simulink model "afe_inv_psm_param"  (R2026b)
settings: Solver=ode23t  StopTime=param.sim.simlength  FixedStep=tc  MaxStep=param.glb_time.tc  RelTol=1e-4
values from neighbouring files (symbols this model uses):
  param = add_template_extras(param, options)    [init_model.m]
undefined symbols (not defined in the file or in its folder): magnitude, omega_m_bez
libraries: fl_lib x330, nesl_utility x174, igbt_simple_2th_lib x12, moving_average_filter x10, moving_average_filter_cc x8, sl_discontinuities x3, single_phase_transformer_lib x3, linear_double_integrator_observer_ccaller x2, discrete_time_low_pass_filter x2, threephase_inductor_lib x2, three_phase_pwm_modulator x2, three_phase_inverter_ideal_switch_based_model x2
(part 7 of 13)

== system afe_inv_psm_param/afe_abc_inv_psm_mod1/AFE_control/afe_control/grid_current_sequences_and_reactive_pwr_ctrl/sequences_current_control/Positive-Seq. eta-Control ==
  ff : Inport
  e : Inport  Port=2
  1/Ti : Gain  Gain=param.afe.ctrl.kp_rc_pos_grid  SaturateOnIntegerOverflow=on  OutDataTypeStr=Inherit: Same as input  ParamDataTypeStr=Inherit: Same as input
  Saturation : Saturate  UpperLimit=param.afe.ctrl.ieta_pos_ref_lim  LowerLimit=-param.afe.ctrl.ieta_pos_ref_lim
  Sum : Sum  Inputs=|++
  Sum2 : Sum  Inputs=+++  SaturateOnIntegerOverflow=on
  Sum3 : Sum  Inputs=-+  SaturateOnIntegerOverflow=on
  Unit Delay4 : UnitDelay  SampleTime=-1
  kp : Gain  Gain=param.afe.ctrl.ki_rc_pos_grid*param.glb_time.ts_afe  SaturateOnIntegerOverflow=on  OutDataTypeStr=Inherit: Same as input  ParamDataTypeStr=Inherit: Same as input
  u : Outport  VectorParamsAs1DForOutWhenUnconnected=off
  wires:
  Unit Delay4/1 -> Sum2/3
  Sum3/1 -> Unit Delay4/1
  kp/1 -> Sum2/2
  Sum2/1 -> Saturation/1
  1/Ti/1 -> Sum2/1, Sum3/1
  Saturation/1 -> Sum/1, Sum3/2
  Sum/1 -> u/1
  e/1 -> 1/Ti/1, kp/1  "e"
  ff/1 -> Sum/2

== system afe_inv_psm_param/afe_abc_inv_psm_mod1/AFE_control/afe_control/grid_voltage_phase_lock_loops/FHT-PLL/pll_stageA ==
  gamma_grid : Inport
  ug_abc_pu : Inport  Port=2
  Demux : Demux  Outputs=3
  Math Function : Math  Operator=magnitude^2  SignedPower=on
  Math Function1 : Math  Operator=magnitude^2  SignedPower=on
  Reciprocal Sqrt : Sqrt  Operator=rSqrt
  Saturation : Saturate  UpperLimit=inf  LowerLimit=0.02
  Sum : Sum  Inputs=|++
  filter_and_transformation : Subsystem
  sequences : Subsystem
  u_grid_xi : Outport  VectorParamsAs1DForOutWhenUnconnected=off
  u_grid_eta : Outport  Port=2  VectorParamsAs1DForOutWhenUnconnected=off
  tag scope: Vgrid_unorm_fht=scoped
  wires:
  gamma_grid/1 -> sequences/3(phase_angle)
  sequences/2(u_grid_eta) -> u_grid_eta/1
  sequences/1(u_grid_xi) -> u_grid_xi/1
  ug_abc_pu/1 -> Demux/1
  Demux/1 -> filter_and_transformation/1(ug_a)
  Demux/2 -> filter_and_transformation/2(ug_b)
  Demux/3 -> filter_and_transformation/3(ug_c)
  filter_and_transformation/1(ug_alpha) -> Math Function/1, sequences/1(u_grid_alpha)
  filter_and_transformation/2(ug_beta) -> Math Function1/1, sequences/2(u_grid_beta)
  Math Function/1 -> Sum/1
  Math Function1/1 -> Sum/2
  Sum/1 -> Saturation/1
  Reciprocal Sqrt/1 -> [Vgrid_unorm_fht]
  Saturation/1 -> Reciprocal Sqrt/1

== system afe_inv_psm_param/afe_abc_inv_psm_mod1/AFE_control/afe_control/grid_voltage_phase_lock_loops/FHT-PLL/pll_stageB ==
  u_grid_pos_xi : Inport
  u_grid_pos_eta : Inport  Port=2
  Constant4 : Constant  Value=param.grid.emu.omega_grid_nom
  Gain : Gain  Gain=-1
  Product : Product  RndMeth=Zero
  Product1 : Product  RndMeth=Zero
  Product2 : Product  RndMeth=Zero
  Sum3 : Sum  SaturateOnIntegerOverflow=on
  Sum4 : Sum  SaturateOnIntegerOverflow=on
  Sum5 : Sum  Inputs=++|
  Terminator : Terminator
  Unit Delay1 : UnitDelay  SampleTime=-1
  Unit Delay2 : UnitDelay  SampleTime=-1
  Unit Delay4 : UnitDelay  SampleTime=-1
  bounder1 : MATLAB Function  TreatAsAtomicUnit=on
  double_integrator_observer : Subsystem
  kp : Gain  Gain=param.afe.ctrl.pll_i1_fht*param.glb_time.ts_afe  SaturateOnIntegerOverflow=on  OutDataTypeStr=Inherit: Same as input  ParamDataTypeStr=Inherit: Same as input
  kp1 : Gain  Gain=param.afe.ctrl.pll_p_fht  SaturateOnIntegerOverflow=on  OutDataTypeStr=Inherit: Same as input  ParamDataTypeStr=Inherit: Same as input
  kp2 : Gain  Gain=param.glb_time.ts_afe  SaturateOnIntegerOverflow=on  OutDataTypeStr=Inherit: Same as input  ParamDataTypeStr=Inherit: Same as input
  kp3 : Gain  Gain=1/param.grid.emu.omega_grid_nom  SaturateOnIntegerOverflow=on  OutDataTypeStr=Inherit: Same as input  ParamDataTypeStr=Inherit: Same as input
  gamma_grid_ddsrf_pll : Outport  VectorParamsAs1DForOutWhenUnconnected=off
  omega_grid_ddsrf_pll : Outport  Port=2  VectorParamsAs1DForOutWhenUnconnected=off
  wires:
  Gain/1 -> kp/1, kp1/1
  Product1/1 -> Gain/1
  kp3/1 -> omega_grid_ddsrf_pll/1
  Product/1 -> Terminator/1
  double_integrator_observer/1(omega_hat) -> kp3/1
  Unit Delay4/1 -> Sum3/2
  Sum4/1 -> bounder1/1(u)
  Unit Delay1/1 -> Sum4/2
  Sum3/1 -> Sum5/2, Unit Delay4/1  "i1"
  kp2/1 -> Sum4/1
  Constant4/1 -> Product2/2
  [Vgrid_unorm_fht] -> Product/2, Product1/2
  kp/1 -> Sum3/1
  Sum5/1 -> Product2/1
  bounder1/1(y) -> Unit Delay2/1, Unit Delay1/1
  u_grid_pos_xi/1 -> Product/1
  u_grid_pos_eta/1 -> Product1/1
  Product2/1 -> kp2/1
  kp1/1 -> Sum5/1
  Unit Delay2/1 -> double_integrator_observer/1(theta), gamma_grid_ddsrf_pll/1

== system afe_inv_psm_param/afe_abc_inv_psm_mod1/AFE_control/afe_control/grid_voltage_phase_lock_loops/FHT-PLL_simulink/pll_stageA ==
  gamma_grid : Inport
  ug_abc_pu : Inport  Port=2
  Demux : Demux  Outputs=3
  Math Function : Math  Operator=magnitude^2  SignedPower=on
  Math Function1 : Math  Operator=magnitude^2  SignedPower=on
  Reciprocal Sqrt : Sqrt  Operator=rSqrt
  Saturation : Saturate  UpperLimit=inf  LowerLimit=0.02
  Sum : Sum  Inputs=|++
  filter_and_transformation : Subsystem
  sequences : Subsystem
  u_grid_xi : Outport  VectorParamsAs1DForOutWhenUnconnected=off
  u_grid_eta : Outport  Port=2  VectorParamsAs1DForOutWhenUnconnected=off
  tag scope: Vgrid_unorm_fht_simulink=scoped
  wires:
  Saturation/1 -> Reciprocal Sqrt/1
  Reciprocal Sqrt/1 -> [Vgrid_unorm_fht_simulink]
  Sum/1 -> Saturation/1
  Math Function1/1 -> Sum/2
  Math Function/1 -> Sum/1
  filter_and_transformation/2(ug_beta) -> sequences/2(u_grid_beta), Math Function1/1
  filter_and_transformation/1(ug_alpha) -> sequences/1(u_grid_alpha), Math Function/1
  Demux/3 -> filter_and_transformation/3(ug_c)
  Demux/2 -> filter_and_transformation/2(ug_b)
  Demux/1 -> filter_and_transformation/1(ug_a)
  ug_abc_pu/1 -> Demux/1
  sequences/1(u_grid_xi) -> u_grid_xi/1
  sequences/2(u_grid_eta) -> u_grid_eta/1
  gamma_grid/1 -> sequences/3(phase_angle)

== system afe_inv_psm_param/afe_abc_inv_psm_mod1/AFE_control/afe_control/grid_voltage_phase_lock_loops/FHT-PLL_simulink/pll_stageB ==
  u_grid_pos_xi : Inport
  u_grid_pos_eta : Inport  Port=2
  Constant4 : Constant  Value=param.grid.emu.omega_grid_nom
  Gain : Gain  Gain=-1
  Product : Product  RndMeth=Zero
  Product1 : Product  RndMeth=Zero
  Product2 : Product  RndMeth=Zero
  Sum3 : Sum  SaturateOnIntegerOverflow=on
  Sum4 : Sum  SaturateOnIntegerOverflow=on
  Sum5 : Sum  Inputs=++|
  Terminator : Terminator
  Unit Delay1 : UnitDelay  SampleTime=-1
  Unit Delay2 : UnitDelay  SampleTime=-1
  Unit Delay4 : UnitDelay  SampleTime=-1
  bounder1 : MATLAB Function  TreatAsAtomicUnit=on
  double_integrator_observer : Subsystem
  kp : Gain  Gain=param.afe.ctrl.pll_i1_fht*param.glb_time.ts_afe  SaturateOnIntegerOverflow=on  OutDataTypeStr=Inherit: Same as input  ParamDataTypeStr=Inherit: Same as input
  kp1 : Gain  Gain=param.afe.ctrl.pll_p_fht  SaturateOnIntegerOverflow=on  OutDataTypeStr=Inherit: Same as input  ParamDataTypeStr=Inherit: Same as input
  kp2 : Gain  Gain=param.glb_time.ts_afe  SaturateOnIntegerOverflow=on  OutDataTypeStr=Inherit: Same as input  ParamDataTypeStr=Inherit: Same as input
  kp3 : Gain  Gain=1/param.grid.emu.omega_grid_nom  SaturateOnIntegerOverflow=on  OutDataTypeStr=Inherit: Same as input  ParamDataTypeStr=Inherit: Same as input
  gamma_grid_ddsrf_pll : Outport  VectorParamsAs1DForOutWhenUnconnected=off
  omega_grid_ddsrf_pll : Outport  Port=2  VectorParamsAs1DForOutWhenUnconnected=off
  wires:
  Unit Delay2/1 -> gamma_grid_ddsrf_pll/1, double_integrator_observer/1(theta)
  kp1/1 -> Sum5/1
  Product2/1 -> kp2/1
  u_grid_pos_eta/1 -> Product1/1
  u_grid_pos_xi/1 -> Product/1
  bounder1/1(y) -> Unit Delay1/1, Unit Delay2/1
  Sum5/1 -> Product2/1
  kp/1 -> Sum3/1
  [Vgrid_unorm_fht_simulink] -> Product1/2, Product/2
  Constant4/1 -> Product2/2
  kp2/1 -> Sum4/1
  Sum3/1 -> Unit Delay4/1, Sum5/2  "i1"
  Unit Delay1/1 -> Sum4/2
  Sum4/1 -> bounder1/1(u)
  Unit Delay4/1 -> Sum3/2
  double_integrator_observer/1(omega_hat) -> kp3/1
  Product/1 -> Terminator/1
  kp3/1 -> omega_grid_ddsrf_pll/1
  Product1/1 -> Gain/1
  Gain/1 -> kp1/1, kp/1

== system afe_inv_psm_param/afe_abc_inv_psm_mod1/AFE_control/afe_control/grid_voltage_phase_lock_loops/dq_pll/pll_stageA ==
  phase_grid : Inport
  ug_abc : Inport  Port=2
  Demux : Demux  Outputs=3
  Math Function : Math  Operator=magnitude^2  SignedPower=on
  Math Function1 : Math  Operator=magnitude^2  SignedPower=on
  Reciprocal Sqrt : Sqrt  Operator=rSqrt
  Saturation : Saturate  UpperLimit=inf  LowerLimit=0.02
  Sum : Sum  Inputs=|++
  mormalization_and_transformation : Subsystem
  sequences : Subsystem
  u_grid_pos_xi : Outport  VectorParamsAs1DForOutWhenUnconnected=off
  u_grid_pos_eta : Outport  Port=2  VectorParamsAs1DForOutWhenUnconnected=off
  tag scope: Vgrid_unorm_dqpll=scoped
  wires:
  ug_abc/1 -> Demux/1
  Demux/1 -> mormalization_and_transformation/1(ug_a)
  Demux/2 -> mormalization_and_transformation/2(ug_b)
  Demux/3 -> mormalization_and_transformation/3(ug_c)
  phase_grid/1 -> sequences/3(gamma_grid)
  sequences/1(u_grid_pos_xi) -> u_grid_pos_xi/1
  sequences/2(u_grid_pos_eta) -> u_grid_pos_eta/1
  Math Function1/1 -> Sum/2
  mormalization_and_transformation/1(ug_alpha) -> Math Function/1, sequences/1(u_grid_alpha)
  mormalization_and_transformation/2(ug_beta) -> Math Function1/1, sequences/2(u_grid_beta)
  Reciprocal Sqrt/1 -> [Vgrid_unorm_dqpll]
  Sum/1 -> Saturation/1
  Math Function/1 -> Sum/1
  Saturation/1 -> Reciprocal Sqrt/1

== system afe_inv_psm_param/afe_abc_inv_psm_mod1/AFE_control/afe_control/grid_voltage_phase_lock_loops/dq_pll/pll_stageB ==
  u_grid_pos_xi : Inport
  u_grid_pos_eta : Inport  Port=2
  -2<x<2 : Saturate  UpperLimit=2  LowerLimit=-2
  Constant4 : Constant  Value=param.grid.emu.omega_grid_nom
  Gain : Gain  Gain=1/param.grid.emu.omega_grid_nom
  Product1 : Product  RndMeth=Zero
  Product2 : Product  RndMeth=Zero
  Sum3 : Sum  SaturateOnIntegerOverflow=on
  Sum4 : Sum  SaturateOnIntegerOverflow=on
  Sum5 : Sum  Inputs=++|
  Terminator : Terminator
  Unit Delay1 : UnitDelay  SampleTime=-1
  Unit Delay2 : UnitDelay  SampleTime=-1
  Unit Delay4 : UnitDelay  SampleTime=-1
  bounder1 : MATLAB Function  TreatAsAtomicUnit=on
  double_integrator_observer : Subsystem
  kp : Gain  Gain=param.afe.ctrl.pll_i1*param.glb_time.ts_afe  SaturateOnIntegerOverflow=on  OutDataTypeStr=Inherit: Same as input  ParamDataTypeStr=Inherit: Same as input
  kp2 : Gain  Gain=param.glb_time.ts_afe  SaturateOnIntegerOverflow=on  OutDataTypeStr=Inherit: Same as input  ParamDataTypeStr=Inherit: Same as input
  scheduled-p-gain : Subsystem
      settings: PortSchema="{\"entries\":[{\"content\":{\"sides\":[{\"content\":{},\"type\":\"ConnectorPlacement.EquallySpacedRectSide\",\"uuid\":\"88e64df2-a299-4c1b-9bac-7a615cd04a00\"},{\"content\":{\"side\":\"RIGHT\"},\"type\":\"ConnectorPlacement.EquallySpacedRectSide\",\"uuid\":\"ef1d7318-b0e2-4e96-bf99-c42bb4ec5202\"},{\"content\":{\"connectorIds\":[\"In1\"],\"side\":\"TOP\"},\"type\":\"ConnectorPlacement.EquallySpacedRectSide\",\"uuid\":\"96582c59-f6c8-40f1-b3cf-394cc239c4b2\"},{\"content\":{\"connectorIds\":[\"Out1\"],\"side\":\"BOTTOM\"},\"type\":\"ConnectorPlacement.EquallySpacedRectSide\",\"uuid\":\"9ac5cd0d-958f-4b67-b4ea-90856a0aa038\"}]},\"type\":\"ConnectorPlacement.EquallySpacedConnector\",\"uuid\":\"ca37db80-6b94-4315-bd9c-66307567cd1f\"}],\"packageUris\":[\"http://schema.mathworks.com/mf0/Connector/R2020b\"],\"version\":\"1.0\"}"
  phase_grid_pll : Outport  VectorParamsAs1DForOutWhenUnconnected=off
  omega_grid_pu_pll : Outport  Port=2  VectorParamsAs1DForOutWhenUnconnected=off
  wires:
  Unit Delay4/1 -> Sum3/2
  Sum3/1 -> -2<x<2/1
  Sum4/1 -> bounder1/1(u)
  Unit Delay1/1 -> Sum4/2
  -2<x<2/1 -> Sum5/2, Unit Delay4/1  "i1"
  kp2/1 -> Sum4/1
  Constant4/1 -> Product2/2
  [Vgrid_unorm_dqpll] -> Product1/2
  kp/1 -> Sum3/1
  Sum5/1 -> Product2/1
  bounder1/1(y) -> Unit Delay1/1, Unit Delay2/1
  u_grid_pos_eta/1 -> Product1/1
  Product2/1 -> kp2/1
  Product1/1 -> scheduled-p-gain/1(In1), kp/1
  scheduled-p-gain/1(Out2) -> Sum5/1
  Unit Delay2/1 -> double_integrator_observer/1(phase), phase_grid_pll/1
  double_integrator_observer/1(omega_hat) -> Gain/1
  Gain/1 -> omega_grid_pu_pll/1
  u_grid_pos_xi/1 -> Terminator/1

== system afe_inv_psm_param/afe_abc_inv_psm_mod1/AFE_control/afe_control/grid_voltage_phase_lock_loops/dq_pll_ccaller/first_harmonic_tracker_phase_u ==
  u : Inport
  Bus Selector : BusSelector  OutputSignals=output_pu_hat
  C Caller : CCaller  FunctionName=first_harmonic_tracker_process_simulink  PortSpecificationStruct="%)30     .    B \\   8    (     @         %    \"     D    !     0         %  0 \"0    $    _    07)G3F%M90  4&]R=$YA;64 4V-O<&4     26YD97@     5'EP90      4VEZ90      27-';&]B86P   X    P    !@    @    $          4    (     0    ,    !         !   P!O=70 #@   #     &    \"     0         !0    @    !     P    $         $  # &]U=  .    .     8    (    !          %    \"     $    &     0         0  ...(+4988 chars)"
  Constant : Constant  Value=param.glb_time.ts_afe
  Constant1 : Constant  Value=0
  Constant4 : Constant  Value=param.afe.ctrl.fht_grid.omega_fht
  Constant5 : Constant  Value=param.afe.ctrl.fht_grid.delta_fht
  Constant6 : Constant  Value=param.afe.ctrl.fht_grid.Ld_fht(1)
  Constant7 : Constant  Value=param.afe.ctrl.fht_grid.Ld_fht(2)
  Data Type Conversion{1..2,6..9} (6 alike) : DataTypeConversion  OutDataTypeStr=single  SaturateOnIntegerOverflow=off  RndMeth=Floor
  Data Type Conversion3 : DataTypeConversion  OutDataTypeStr=uint8  SaturateOnIntegerOverflow=off  RndMeth=Floor
  Data Type Conversion4 : DataTypeConversion  OutDataTypeStr=double  SaturateOnIntegerOverflow=off  RndMeth=Floor
  Data Type Conversion5 : DataTypeConversion  OutDataTypeStr=uint8  SaturateOnIntegerOverflow=off  RndMeth=Floor
  Step : Step  Time=0.0125  InitialValue=1  FinalValue=0
  u_hat : Outport
  wires:
  Data Type Conversion4/1 -> u_hat/1
  Data Type Conversion3/1 -> C Caller/1
  Data Type Conversion1/1 -> C Caller/3
  Data Type Conversion2/1 -> C Caller/2
  C Caller/1 -> Bus Selector/1
  Bus Selector/1 -> Data Type Conversion4/1  "<output_pu_hat>"
  Step/1 -> Data Type Conversion3/1
  u/1 -> Data Type Conversion2/1
  Constant/1 -> Data Type Conversion1/1
  Constant1/1 -> Data Type Conversion5/1
  Constant4/1 -> Data Type Conversion6/1
  Constant6/1 -> Data Type Conversion8/1
  Constant7/1 -> Data Type Conversion9/1
  Constant5/1 -> Data Type Conversion7/1
  Data Type Conversion5/1 -> C Caller/8
  Data Type Conversion6/1 -> C Caller/4
  Data Type Conversion7/1 -> C Caller/5
  Data Type Conversion8/1 -> C Caller/6
  Data Type Conversion9/1 -> C Caller/7

== system afe_inv_psm_param/afe_abc_inv_psm_mod1/AFE_control/afe_control/grid_voltage_phase_lock_loops/dq_pll_ccaller/first_harmonic_tracker_phase_v ==
  u : Inport
  Bus Selector : BusSelector  OutputSignals=output_pu_hat
  C Caller : CCaller  FunctionName=first_harmonic_tracker_process_simulink  PortSpecificationStruct="%)30     .    B \\   8    (     @         %    \"     D    !     0         %  0 \"0    $    _    07)G3F%M90  4&]R=$YA;64 4V-O<&4     26YD97@     5'EP90      4VEZ90      27-';&]B86P   X    P    !@    @    $          4    (     0    ,    !         !   P!O=70 #@   #     &    \"     0         !0    @    !     P    $         $  # &]U=  .    .     8    (    !          %    \"     $    &     0         0  ...(+4988 chars)"
  Constant : Constant  Value=param.glb_time.ts_afe
  Constant1 : Constant  Value=2
  Constant4 : Constant  Value=param.afe.ctrl.fht_grid.omega_fht
  Constant5 : Constant  Value=param.afe.ctrl.fht_grid.delta_fht
  Constant6 : Constant  Value=param.afe.ctrl.fht_grid.Ld_fht(1)
  Constant7 : Constant  Value=param.afe.ctrl.fht_grid.Ld_fht(2)
  Data Type Conversion{1..2,6..9} (6 alike) : DataTypeConversion  OutDataTypeStr=single  SaturateOnIntegerOverflow=off  RndMeth=Floor
  Data Type Conversion3 : DataTypeConversion  OutDataTypeStr=uint8  SaturateOnIntegerOverflow=off  RndMeth=Floor
  Data Type Conversion4 : DataTypeConversion  OutDataTypeStr=double  SaturateOnIntegerOverflow=off  RndMeth=Floor
  Data Type Conversion5 : DataTypeConversion  OutDataTypeStr=uint8  SaturateOnIntegerOverflow=off  RndMeth=Floor
  Step : Step  Time=0.0125  InitialValue=1  FinalValue=0
  u_hat : Outport
  wires:
  Data Type Conversion9/1 -> C Caller/7
  Data Type Conversion8/1 -> C Caller/6
  Data Type Conversion7/1 -> C Caller/5
  Data Type Conversion6/1 -> C Caller/4
  Data Type Conversion5/1 -> C Caller/8
  Constant5/1 -> Data Type Conversion7/1
  Constant7/1 -> Data Type Conversion9/1
  Constant6/1 -> Data Type Conversion8/1
  Constant4/1 -> Data Type Conversion6/1
  Constant1/1 -> Data Type Conversion5/1
  Constant/1 -> Data Type Conversion1/1
  u/1 -> Data Type Conversion2/1
  Step/1 -> Data Type Conversion3/1
  Bus Selector/1 -> Data Type Conversion4/1  "<output_pu_hat>"
  C Caller/1 -> Bus Selector/1
  Data Type Conversion2/1 -> C Caller/2
  Data Type Conversion1/1 -> C Caller/3
  Data Type Conversion3/1 -> C Caller/1
  Data Type Conversion4/1 -> u_hat/1

== system afe_inv_psm_param/afe_abc_inv_psm_mod1/AFE_control/afe_control/grid_voltage_phase_lock_loops/dq_pll_ccaller/first_harmonic_tracker_phase_w ==
  u : Inport
  Bus Selector : BusSelector  OutputSignals=output_pu_hat
  C Caller : CCaller  FunctionName=first_harmonic_tracker_process_simulink  PortSpecificationStruct="%)30     .    B \\   8    (     @         %    \"     D    !     0         %  0 \"0    $    _    07)G3F%M90  4&]R=$YA;64 4V-O<&4     26YD97@     5'EP90      4VEZ90      27-';&]B86P   X    P    !@    @    $          4    (     0    ,    !         !   P!O=70 #@   #     &    \"     0         !0    @    !     P    $         $  # &]U=  .    .     8    (    !          %    \"     $    &     0         0  ...(+4988 chars)"
  Constant : Constant  Value=param.glb_time.ts_afe
  Constant1 : Constant  Value=4
  Constant4 : Constant  Value=param.afe.ctrl.fht_grid.omega_fht
  Constant5 : Constant  Value=param.afe.ctrl.fht_grid.delta_fht
  Constant6 : Constant  Value=param.afe.ctrl.fht_grid.Ld_fht(1)
  Constant7 : Constant  Value=param.afe.ctrl.fht_grid.Ld_fht(2)
  Data Type Conversion{1..2,6..9} (6 alike) : DataTypeConversion  OutDataTypeStr=single  SaturateOnIntegerOverflow=off  RndMeth=Floor
  Data Type Conversion3 : DataTypeConversion  OutDataTypeStr=uint8  SaturateOnIntegerOverflow=off  RndMeth=Floor
  Data Type Conversion4 : DataTypeConversion  OutDataTypeStr=double  SaturateOnIntegerOverflow=off  RndMeth=Floor
  Data Type Conversion5 : DataTypeConversion  OutDataTypeStr=uint8  SaturateOnIntegerOverflow=off  RndMeth=Floor
  Step : Step  Time=0.0125  InitialValue=1  FinalValue=0
  u_hat : Outport
  wires:
  Data Type Conversion4/1 -> u_hat/1
  Data Type Conversion3/1 -> C Caller/1
  Data Type Conversion1/1 -> C Caller/3
  Data Type Conversion2/1 -> C Caller/2
  C Caller/1 -> Bus Selector/1
  Bus Selector/1 -> Data Type Conversion4/1  "<output_pu_hat>"
  Step/1 -> Data Type Conversion3/1
  u/1 -> Data Type Conversion2/1
  Constant/1 -> Data Type Conversion1/1
  Constant1/1 -> Data Type Conversion5/1
  Constant4/1 -> Data Type Conversion6/1
  Constant6/1 -> Data Type Conversion8/1
  Constant7/1 -> Data Type Conversion9/1
  Constant5/1 -> Data Type Conversion7/1
  Data Type Conversion5/1 -> C Caller/8
  Data Type Conversion6/1 -> C Caller/4
  Data Type Conversion7/1 -> C Caller/5
  Data Type Conversion8/1 -> C Caller/6
  Data Type Conversion9/1 -> C Caller/7

== system afe_inv_psm_param/afe_abc_inv_psm_mod1/AFE_control/afe_control/grid_voltage_sequences/voltage_sequence_avg/average_filter ==
  v_grid_pos_xi : Inport
  v_grid_pos_eta : Inport  Port=2
  v_grid_neg_xi : Inport  Port=3
  v_grid_neg_eta : Inport  Port=4
  Abs : Abs  SaturateOnIntegerOverflow=off
  Gain : Gain  Gain=param.grid.emu.omega_grid_nom*param.ctrl.mavarage_filter_frequency_base_order
  Saturation : Saturate  UpperLimit=2  LowerLimit=0.1
  dmavg_flt{,1..3} (4 alike) : moving_average_filter/dmavg_flt  ts=param.glb_time.ts_afe  enable_time=param.ctrl.dmavg_filter_enable_time
  v_grid_pos_xi_avg : Outport
  v_grid_pos_eta_avg : Outport  Port=2
  v_grid_neg_xi_avg : Outport  Port=3
  v_grid_neg_eta_avg : Outport  Port=4
  wires:
  v_grid_neg_eta/1 -> dmavg_flt3/1
  v_grid_neg_xi/1 -> dmavg_flt2/1
  v_grid_pos_eta/1 -> dmavg_flt1/1
  dmavg_flt3/1 -> v_grid_neg_eta_avg/1
  dmavg_flt2/1 -> v_grid_neg_xi_avg/1
  dmavg_flt1/1 -> v_grid_pos_eta_avg/1
  Gain/1 -> dmavg_flt/2, dmavg_flt1/2, dmavg_flt2/2, dmavg_flt3/2
  dmavg_flt/1 -> v_grid_pos_xi_avg/1
  v_grid_pos_xi/1 -> dmavg_flt/1
  Abs/1 -> Saturation/1
  [omega_grid_pll_pu] -> Abs/1
  Saturation/1 -> Gain/1

== system afe_inv_psm_param/afe_abc_inv_psm_mod1/AFE_control/afe_control/grid_voltage_sequences/voltage_sequence_avg/average_filter_ccaller ==
  v_grid_pos_xi : Inport
  v_grid_pos_eta : Inport  Port=2
  v_grid_neg_xi : Inport  Port=3
  v_grid_neg_eta : Inport  Port=4
  Abs : Abs  SaturateOnIntegerOverflow=off
  Gain : Gain  Gain=param.grid.emu.omega_grid_nom*param.ctrl.mavarage_filter_frequency_base_order
  Saturation : Saturate  UpperLimit=2  LowerLimit=0.1
  dmavg_flt : moving_average_filter_cc/dmavg_flt  instance=0  ts=param.glb_time.ts_afe  enable_time=param.ctrl.dmavg_filter_enable_time
  dmavg_flt1 : moving_average_filter_cc/dmavg_flt  instance=1  ts=param.glb_time.ts_afe  enable_time=param.ctrl.dmavg_filter_enable_time
  dmavg_flt2 : moving_average_filter_cc/dmavg_flt  instance=2  ts=param.glb_time.ts_afe  enable_time=param.ctrl.dmavg_filter_enable_time
  dmavg_flt3 : moving_average_filter_cc/dmavg_flt  instance=3  ts=param.glb_time.ts_afe  enable_time=param.ctrl.dmavg_filter_enable_time
  v_grid_pos_xi_avg : Outport
  v_grid_pos_eta_avg : Outport  Port=2
  v_grid_neg_xi_avg : Outport  Port=3
  v_grid_neg_eta_avg : Outport  Port=4
  wires:
  v_grid_pos_xi/1 -> dmavg_flt/1
  dmavg_flt/1 -> v_grid_pos_xi_avg/1
  dmavg_flt1/1 -> v_grid_pos_eta_avg/1
  dmavg_flt2/1 -> v_grid_neg_xi_avg/1
  dmavg_flt3/1 -> v_grid_neg_eta_avg/1
  v_grid_pos_eta/1 -> dmavg_flt1/1
  v_grid_neg_xi/1 -> dmavg_flt2/1
  v_grid_neg_eta/1 -> dmavg_flt3/1
  Abs/1 -> Saturation/1
  Saturation/1 -> Gain/1
  [omega_grid_pll_pu] -> Abs/1
  Gain/1 -> dmavg_flt/2, dmavg_flt1/2, dmavg_flt3/2, dmavg_flt2/2

== system afe_inv_psm_param/afe_abc_inv_psm_mod1/AFE_control/afe_control/phase_compensation_1/alignment_eval_afe1/pi ==
  u_ref : Inport
  u : Inport  Port=2
  1/Ti : Gain  Gain=kp  SaturateOnIntegerOverflow=on  OutDataTypeStr=Inherit: Same as input  ParamDataTypeStr=Inherit: Same as input
  Saturation : Saturate  UpperLimit=lim_up  LowerLimit=lim_down
  Sum1 : Sum  Inputs=+++  SaturateOnIntegerOverflow=on
  Sum2 : Sum  Inputs=-+  SaturateOnIntegerOverflow=on
  Sum3 : Sum  Inputs=-+  SaturateOnIntegerOverflow=on
  Unit Delay4 : UnitDelay  SampleTime=-1
  kp : Gain  Gain=ki  SaturateOnIntegerOverflow=on  OutDataTypeStr=Inherit: Same as input  ParamDataTypeStr=Inherit: Same as input
  y : Outport
  wires:
  1/Ti/1 -> Sum1/1, Sum3/1
  kp/1 -> Sum1/2
  Sum3/1 -> Unit Delay4/1
  Unit Delay4/1 -> Sum1/3
  u_ref/1 -> Sum2/2
  u/1 -> Sum2/1
  Sum2/1 -> kp/1, 1/Ti/1
  Sum1/1 -> Saturation/1
  Saturation/1 -> Sum3/2, y/1

== system afe_inv_psm_param/afe_abc_inv_psm_mod1/INV_control/inverter_control/current_ctrl/bemf_observer/EKF_bemf_observer ==
  ialpha_pu : Inport
  ibeta_pu : Inport  Port=2
  ualpha_pu : Inport  Port=3
  ubeta_pu : Inport  Port=4
  udc_pu : Inport  Port=5
  EKF Observer simulink/Ccaller mod1 : Scope  NumInputPorts=2
      settings: ActiveDisplayYMinimum=-3.9268483156565956  ActiveDisplayYMaximum=3.9269848822951774
  Gain : Gain  Gain=param.psm.u_psm_scale_ekf
  Gain1 : Gain  Gain=param.psm.u_psm_scale_ekf
  Mux{,1..3} (4 alike) : Mux  Inputs=2
  Terminator : Terminator
  extended_kalman_observer : Subsystem
  phase_elec_ekf_hat : Outport
  omega_elec_ekf_hat : Outport  Port=2
  tag scope: psi_r_alpha_hat_mod1=scoped, psi_r_beta_hat_mod1=scoped
  wires:
  ialpha_pu/1 -> Mux2/1
  ibeta_pu/1 -> Mux2/2
  Mux/1 -> EKF Observer simulink/Ccaller mod1/1
  Mux1/1 -> EKF Observer simulink/Ccaller mod1/2
  extended_kalman_observer/3(phase_elec_ekf_hat) -> phase_elec_ekf_hat/1, Mux1/1  "phase_elec_ekf_hat"
  extended_kalman_observer/4(omega_elec_ekf_hat) -> omega_elec_ekf_hat/1, Mux/1  "omega_elec_ekf_hat"
  [omegad_pu_psm] -> Mux/2  "omega_pu_psm_encoder"
  [phased_psm] -> Mux1/2  "phase_psm_encoder"
  udc_pu/1 -> Terminator/1
  extended_kalman_observer/1(psi_alpha_ekf_hat) -> [psi_r_alpha_hat_mod1]
  extended_kalman_observer/2(psi_beta_ekf_hat) -> [psi_r_beta_hat_mod1]
  Mux2/1 -> extended_kalman_observer/2(ialphabeta)
  Mux3/1 -> extended_kalman_observer/1(ualphabeta)
  Gain/1 -> Mux3/1
  Gain1/1 -> Mux3/2
  ualpha_pu/1 -> Gain/1
  ubeta_pu/1 -> Gain1/1

== system afe_inv_psm_param/afe_abc_inv_psm_mod1/INV_control/inverter_control/current_ctrl/bemf_observer/bemf_observer ==
  ialpha_pu : Inport
  ibeta_pu : Inport  Port=2
  ualpha_pu : Inport  Port=3
  ubeta_pu : Inport  Port=4
  udc_pu : Inport  Port=5
  Gain : Gain  Gain=param.psm.machine.psi_m_norm
  Gain1 : Gain  Gain=param.psm.machine.psi_m_norm
  Goto Tag Visibility : GotoTagVisibility  GotoTag=psi_r_alpha_hat_mod1
  Goto Tag Visibility1 : GotoTagVisibility  GotoTag=psi_r_beta_hat_mod1
  Goto Tag Visibility2 : GotoTagVisibility  GotoTag=theta_bemf_hat_mod1
  Goto Tag Visibility3 : GotoTagVisibility  GotoTag=psi_r_m_alpha_mod1
  Goto Tag Visibility4 : GotoTagVisibility  GotoTag=psi_r_m_beta_mod1
  Trigonometric Function : Trigonometry  Operator=cos
  Trigonometric Function1 : Trigonometry
  double_integrator_observer : Subsystem
  psi_alpha_hat : Subsystem
  psi_beta_hat : Subsystem
  theta_bemf_hat : Subsystem
  omega_pu : Outport
  theta_hat : Outport  Port=2
  tag scope: psi_r_alpha_hat_mod1=scoped, psi_r_alpha_pu_hat_mod1=scoped, psi_r_beta_hat_mod1=scoped, psi_r_beta_pu_hat_mod1=scoped, psi_r_m_alpha_mod1=scoped, psi_r_m_beta_mod1=scoped, theta_bemf_hat_mod1=scoped
  wires:
  Trigonometric Function/1 -> Gain/1
  Trigonometric Function1/1 -> Gain1/1
  ialpha_pu/1 -> psi_alpha_hat/2(ialpha)
  ibeta_pu/1 -> psi_beta_hat/2(ibeta)
  psi_alpha_hat/2(psi_r_alpha_hat) -> [psi_r_alpha_hat_mod1]
  psi_beta_hat/2(psi_r_beta_hat) -> [psi_r_beta_hat_mod1]
  [psi_r_alpha_hat_mod1] -> theta_bemf_hat/1(psi_r_alpha_hat)
  [psi_r_beta_hat_mod1] -> theta_bemf_hat/2(psi_r_beta_hat)
  ualpha_pu/1 -> psi_alpha_hat/1(ualpha)
  ubeta_pu/1 -> psi_beta_hat/1(ubeta)
  [phase_hat_mod1] -> Trigonometric Function/1, Trigonometric Function1/1
  Gain/1 -> [psi_r_m_alpha_mod1]
  Gain1/1 -> [psi_r_m_beta_mod1]
  theta_bemf_hat/1(theta_emf_hat) -> [theta_bemf_hat_mod1]
  [theta_bemf_hat_mod1] -> double_integrator_observer/1(theta)
  double_integrator_observer/1(omega_pu_hat) -> omega_pu/1
  double_integrator_observer/2(theta_hat) -> theta_hat/1
  [psi_r_alpha_hat_mod1] -> [psi_r_alpha_pu_hat_mod1]
  [psi_r_beta_hat_mod1] -> [psi_r_beta_pu_hat_mod1]
  udc_pu/1 -> psi_alpha_hat/3(udc), psi_beta_hat/3(udc)
